simulink model "gnc_PathAnalyzer"  (R2026b)
settings: Solver=VariableStepAuto
values from neighbouring files (symbols this model uses):
  Ts = prm.Ts    [gnc_missionFSM.m]    (also in gnc_mpcPlantUpdate.m)
undefined symbols (not defined in the file or in its folder): P
settings Model: Creator=aomar  LastModifiedBy=aomar

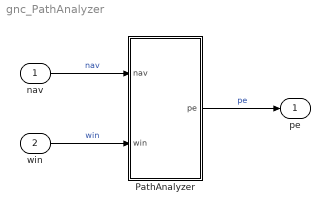
== system gnc_PathAnalyzer ==
  nav : Inport  OutDataTypeStr=Bus: Bus_NavCond  SampleTime=Ts.gnc
  win : Inport  Port=2  OutDataTypeStr=Bus: Bus_PathWindow  SampleTime=Ts.gnc
  PathAnalyzer : MATLAB Function  TreatAsAtomicUnit=on  mask{pa=P.gnc.pa}
  pe : Outport  OutDataTypeStr=Bus: Bus_PathError
  wires:
  nav/1 -> PathAnalyzer/1(nav)  "nav"
  win/1 -> PathAnalyzer/2(win)  "win"
  PathAnalyzer/1(pe) -> pe/1  "pe"

== matlab function gnc_PathAnalyzer/PathAnalyzer ==
  settings: updateMethod=DISCRETE  sampleTime=Ts.gnc  description=Closest point, cross-track / heading error, progress, curvature preview (gnc spec 4.2); body subsystems/gnc/gnc_pathAnalyzer.m.
  data: nav input Bus: Bus_NavCond; pe output Bus: Bus_PathError; win input Bus: Bus_PathWindow; pa parameter
function pe = fcn(nav, win, pa)
%#codegen
pe = gnc_pathAnalyzer(nav, win, pa);
